simulink library "Smoothers"  (R2012a)
settings: Solver=ode45  StartTime=0.0  StopTime=10.0  RelTol=1e-3
settings Model: CovSaveCumulativeToWorkspaceVar=on  Creator=admin  LastModifiedBy=admin

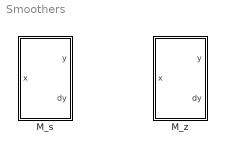
== system Smoothers ==
  M_s : Subsystem  mask{T=1, Q0=0}
      mask prompts: T "T_i"; Q0 "Initial Condition"
  M_z : Subsystem  mask{N=100, Ts=1, Q0=0}
      mask prompts: N "N_i"; Ts "Sampling period (Ts)"; Q0 "Initial position"

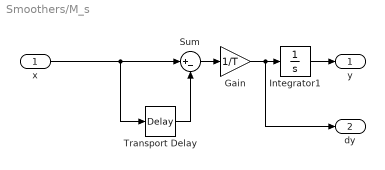
== system Smoothers/M_s ==
  x : Inport
  Gain : Gain  Gain=1/T
  Integrator1 : Integrator  InitialCondition=Q0
  Sum : Sum  Inputs=|+-
  Transport Delay : TransportDelay  DelayTime=T  InitialOutput=Q0  BufferSize=10000
  y : Outport
  dy : Outport  Port=2
  wires:
  Integrator1/1 -> y/1
  Gain/1 -> Integrator1/1, dy/1
  x/1 -> Transport Delay/1, Sum/1
  Transport Delay/1 -> Sum/2
  Sum/1 -> Gain/1

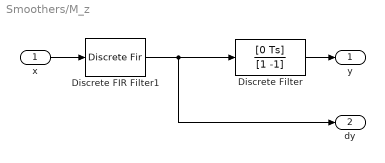
== system Smoothers/M_z ==
  x : Inport
  Discrete FIR Filter1 : DiscreteFir  Coefficients=1/N/Ts*[1 zeros(1,N-1) -1]  InitialStates=Q0  SampleTime=Ts
  Discrete Filter : DiscreteFilter  Numerator=[0 Ts]  Denominator=[1 -1]  InitialStates=Q0  SampleTime=Ts
  y : Outport
  dy : Outport  Port=2
  wires:
  Discrete Filter/1 -> y/1
  x/1 -> Discrete FIR Filter1/1
  Discrete FIR Filter1/1 -> dy/1, Discrete Filter/1
